simulink model "tema_lunga"  (R2024b)
settings: Solver=VariableStepAuto  StartTime=0.0  StopTime=10.0  RelTol=1e-3
settings Model: Creator=alex_  LastModifiedBy=alex_

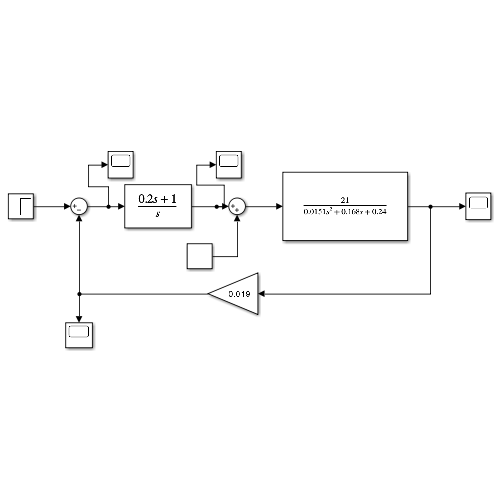
[thumbnail: Simulink's stored preview of the top-level diagram]
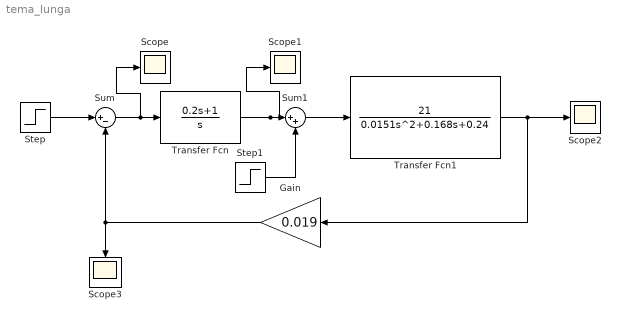
== system tema_lunga ==
  Gain : Gain  Gain=0.019
  Scope{,1..3} (4 alike) : Scope
  Step : Step  Time=4.75  SampleTime=0
  Step1 : Step  Time=500  SampleTime=0
  Sum : Sum  Inputs=|+-
  Sum1 : Sum  Inputs=|++
  Transfer Fcn : TransferFcn  Numerator=[0.2 1]  Denominator=[1 0]
  Transfer Fcn1 : TransferFcn  Numerator=[21]  Denominator=[0.0151 0.168 0.24]
  wires:
  Sum/1 -> Scope/1, Transfer Fcn/1
  Transfer Fcn/1 -> Scope1/1, Sum1/1
  Transfer Fcn1/1 -> Gain/1, Scope2/1
  Gain/1 -> Sum/2, Scope3/1
  Step/1 -> Sum/1
  Step1/1 -> Sum1/2
  Sum1/1 -> Transfer Fcn1/1
